simulink model "DCMOTOR"  (R2026a)
settings: Solver=VariableStepAuto  StopTime=10
model workspace (MAT data in the model file):
  B = 0.0005
  J = 5e-05
  K = 0.2
  L = 0.01
  R = 4
  V = 7.4
settings Model: Creator=ismail  LastModifiedBy=ismail

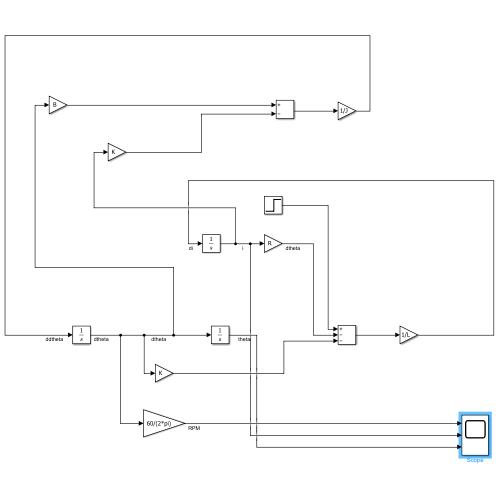
[thumbnail: Simulink's stored preview of the top-level diagram]
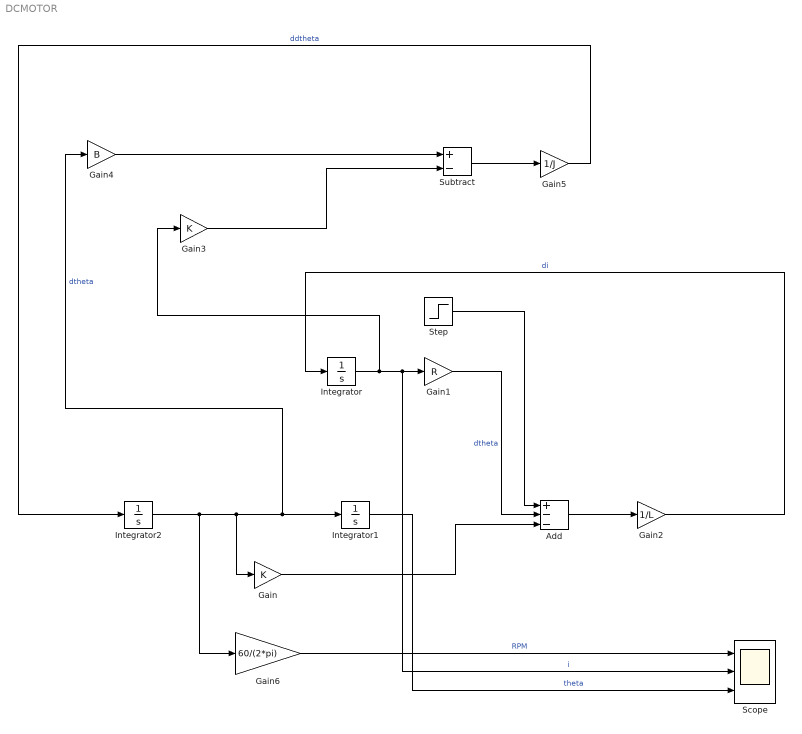
== system DCMOTOR ==
  Add : Sum  Inputs=+--
  Gain : Gain  Gain=K
  Gain1 : Gain  Gain=R
  Gain2 : Gain  Gain=1/L
  Gain3 : Gain  Gain=K
  Gain4 : Gain  Gain=B
  Gain5 : Gain  Gain=1/J
  Gain6 : Gain  Gain=60/(2*pi)
  Integrator : Integrator
  Integrator1 : Integrator
  Integrator2 : Integrator
  Scope : Scope  NumInputPorts=3
      settings: ActiveDisplayYMinimum=-1.0799591628626729E+153  ActiveDisplayYMaximum=2.2002204169197779E+152
  Step : Step  FinalValue=V  SampleTime=0
  Subtract : Sum  Inputs=+-
  wires:
  Gain2/1 -> Integrator/1  "di"
  Integrator/1 -> Gain3/1, Scope/2, Gain1/1  "i"
  Integrator1/1 -> Scope/3  "theta"
  Gain5/1 -> Integrator2/1  "ddtheta"
  Integrator2/1 -> Gain6/1, Gain/1, Gain4/1, Integrator1/1  "dtheta"
  Step/1 -> Add/1
  Gain1/1 -> Add/2  "dtheta"
  Gain/1 -> Add/3
  Add/1 -> Gain2/1
  Gain4/1 -> Subtract/1
  Gain3/1 -> Subtract/2
  Subtract/1 -> Gain5/1
  Gain6/1 -> Scope/1  "RPM"
